simulink model "robot_shooter_test"  (R2023b)
settings: Solver=VariableStepAuto  StartTime=0.0  StopTime=10.0  RelTol=1e-3
settings Model: Creator=hilat  LastModifiedBy=hilat

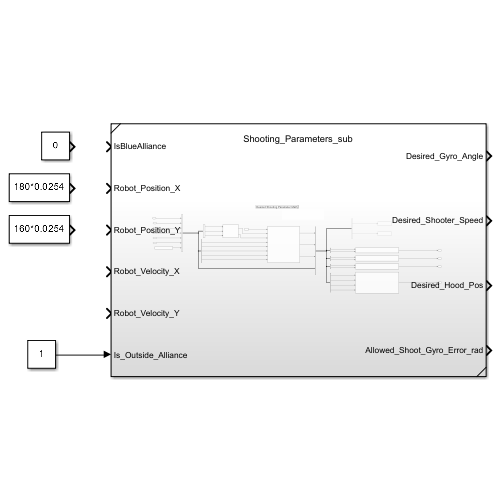
[thumbnail: Simulink's stored preview of the top-level diagram]
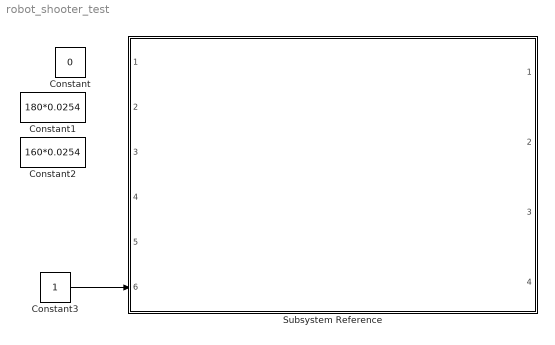
== system robot_shooter_test ==
  Constant : Constant  Value=0
  Constant1 : Constant  Value=180*0.0254
  Constant2 : Constant  Value=160*0.0254
  Constant3 : Constant
  Subsystem Reference : Subsystem  ReferencedSubsystem=Shooting_Parameters_sub
  wires:
  Constant3/1 -> Subsystem Reference/6
